simulink model "foc_can_probe"  (R2023a)
settings: Solver=FixedStepDiscrete  StartTime=0.0  StopTime=inf  FixedStep=0.01  RelTol=1e-3  EnableMultiTasking=on
libraries: c280xlib x3, simulink x1, c2838xlib x1
settings Model: ExtModeTrigDuration=8  Creator=Student  LastModifiedBy=Student
settings OptimizationCC: DefaultUnderspecifiedDataType=single  EnhancedBackFolding=on  PassReuseOutputArgsAs=Individual arguments  MaxStackSize=1024  OptimizeBlockOrder=speed  DifferentSizesBufferReuse=on  OptimizationCustomize=off  DenormalBehavior=FlushToZero  EfficientTunableParamExpr=on
settings DebuggingCC: ParameterTunabilityLossMsg=error
settings HardwareCC: ProdBitPerChar=16  ProdBitPerInt=16  ProdBitPerPointer=32  ProdBitPerSizeT=32  ProdBitPerPtrDiffT=32  ProdLargestAtomicInteger=Integer  ProdLargestAtomicFloat=None  ProdWordSize=16  ProdLongLongMode=on  ProdHWDeviceType=Texas Instruments->C2000  HardwareBoardFeatureSet=SoCBlockset
settings ModelReferenceCC: ModelReferenceNumInstancesAllowed=Single
settings SFSimCC: MATLABDynamicMemAlloc=off
settings RTWCC: Description=Embedded Coder  SystemTargetFile=ert.tlc  HardwareBoard=TI F2838x  TemplateMakefile=ert_default_tmf  Toolchain=Texas Instruments Code Composer Studio - EABI (C2000)
settings CodeAppCC: ForceParamTrailComments=on  IgnoreCustomStorageClasses=off  OperatorAnnotations=on  SimulinkDataObjDesc=on  SFDataObjDesc=on  InsertBlockDesc=on
settings ERTTargetCC: CodeReplacementLibrary=TI C28x  ExtModeTransport=4  ExtModeStaticAlloc=on  ExtModeAutomaticAllocSize=off  ExtModeStaticAllocSize=10000  ExtModeMexFile=ext_xcp  ExtModeIntrfLevel=Level2 - Open

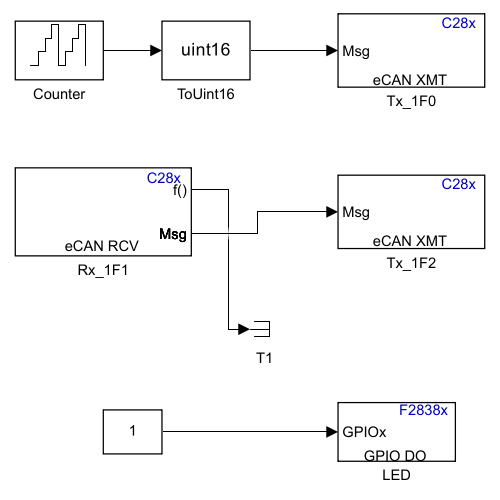
[thumbnail: Simulink's stored preview of the top-level diagram]
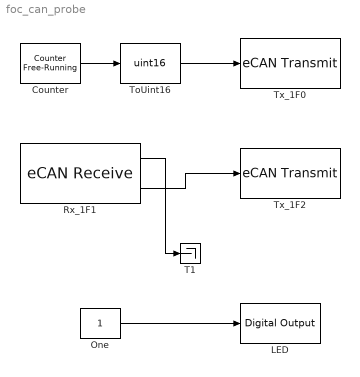
== system foc_can_probe ==
  Counter : simulink/Sources/Counter Free-Running  NumBits=16  tsamp=0.2
  LED : c2838xlib/Digital Output  GPIO_Number=GPIO56~GPIO63  GPIO_Bit0=on  GPIO_BIT0_Toggle=on  GPIO_Bit1=off  GPIO_BIT1_Toggle=off  GPIO_Bit2=off  GPIO_BIT2_Toggle=off  GPIO_Bit3=off  GPIO_BIT3_Toggle=off  GPIO_Bit4=off  GPIO_BIT4_Toggle=off  GPIO_Bit5=off  GPIO_BIT5_Toggle=off  GPIO_Bit6=off  GPIO_BIT6_Toggle=off  GPIO_Bit7=off  GPIO_BIT7_Toggle=off
  One : Constant  OutDataTypeStr=boolean  SampleTime=0.25
  Rx_1F1 : c280xlib/eCAN Receive  chipFamily=C280x  useModule=eCAN_A  mailboxNo=9  messageID=hex2dec('1F1')  messageType=Standard (11-bit identifier)  enableAcceptanceFiltering=off  messageIDMask=0  sampleTime=0.2  dataType=uint16  outputAction=Output last received values  initValue=0  outputMessageID=off  outputMessageLength=off  outputMessageTimeStamp=off  postInterrupt=off  interruptLine=0
      settings: LibrarySourceBlock=c2838xlib/eCAN Receive
  T1 : Terminator
  ToUint16 : DataTypeConversion  OutDataTypeStr=uint16  SaturateOnIntegerOverflow=off  RndMeth=Floor
  Tx_1F0 : c280xlib/eCAN Transmit  chipFamily=C280x  useModule=eCAN_A  mailboxNo=1  messageID=hex2dec('1F0')  messageType=Standard (11-bit identifier)  enableBlockingMode=off  postInterrupt=off  interruptLine=0
      settings: LibrarySourceBlock=c2838xlib/eCAN Transmit
  Tx_1F2 : c280xlib/eCAN Transmit  chipFamily=C280x  useModule=eCAN_A  mailboxNo=2  messageID=hex2dec('1F2')  messageType=Standard (11-bit identifier)  enableBlockingMode=off  postInterrupt=off  interruptLine=0
      settings: LibrarySourceBlock=c2838xlib/eCAN Transmit
  wires:
  Counter/1 -> ToUint16/1
  ToUint16/1 -> Tx_1F0/1
  Rx_1F1/2 -> Tx_1F2/1
  Rx_1F1/1 -> T1/1
  One/1 -> LED/1
